simulink model "SC03_testbench"  (R2025a)
settings: Solver=ode23tb  StartTime=0.0  StopTime=52.6667  MaxStep=1e-5  RelTol=1e-4
InitFcn:
  | tbModel = 'SC03_testbench'; sc03_tb_init
model workspace (MAT data in the model file):
  tbGroup = 'bat'
values from neighbouring files (symbols this model uses):
  sw = swMap_(cfg)    [sc03_tb_init.m]
  useMem = double(cfg == 4)    [sc03_tb_init.m]
undefined symbols (not defined in the file or in its folder): Ion, Lithium, scen
libraries: spsSeriesRLCBranchLib x8, spsDiodeLib x4, spsPVArrayLib x4, simulink x3, spsCurrentMeasurementLib x2, fuzblock x2, spsBatteryLib x1, spsBuckConverterLib x1, spsGroundLib x1, spsVoltageMeasurementLib x1, sps_lib x1
settings Model: PauseTimes=8  Creator=kaush  LastModifiedBy=kaush
settings SolverCC: ZeroCrossAlgorithm=Adaptive  AlgebraicLoopSolver=TrustRegion
settings DataIOCC: SignalLogging=off
settings DebuggingCC: AlgebraicLoopMsg=none  IgnoredZcDiagnostic=none

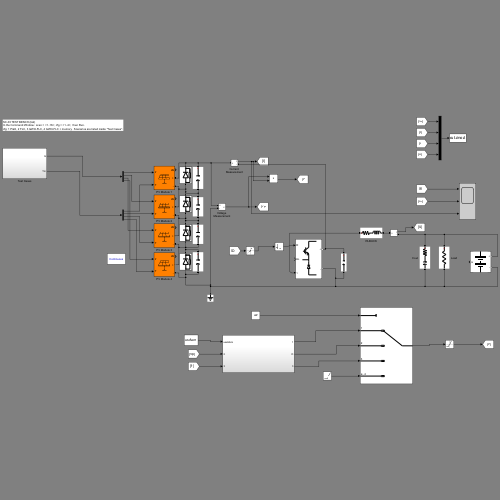
[thumbnail: Simulink's stored preview of the top-level diagram]
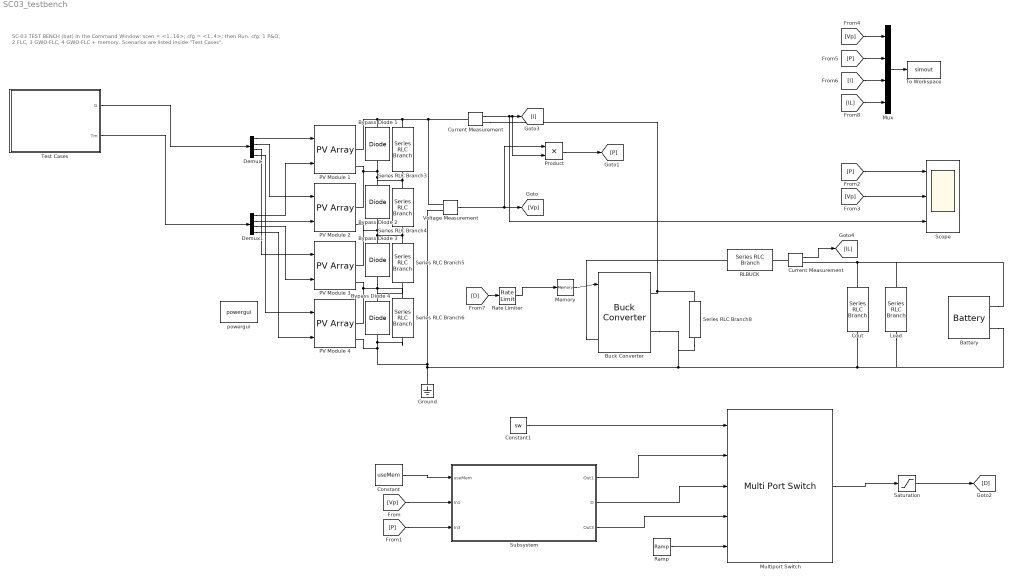
== system SC03_testbench ==
  note: SC-03 TEST BENCH (bat)
      | In the Command Window:  scen = <1..16>; cfg = <1..4>;  then Run.
      | cfg: 1 P&O, 2 FLC, 3 GWO-FLC, 4 GWO-FLC + memory.  Scenarios are listed inside "Test Cases".
  Battery : spsBatteryLib/Battery  BatType=Lithium-Ion  NomV=12.8  NomQ=160  SOC=55  Batt_Tr=30  PresetModel=off  MaxQ=160  MinV=11.2  FullV=14.4  Dis_rate=69.5652  R=0.0009  Normal_OP=144.6957  expZone="[13.8289      7.86087]"
  Buck Converter : spsBuckConverterLib/Buck Converter  ModelType=Average model (D-controlled)  Ron=1e-3  Rs=1e6  Cs=inf  Vforward=[0,0]  Ron_Diode=1e-3  Rs_Diode=1e6  Cs_Diode=inf  Vf_Diode=1e-3  Rs_CurrentSource=inf  Ron_ACsource=1e-3
      settings: LibrarySourceBlock=sps_lib/Power Electronics/Buck Converter
  Bypass Diode {1..4} (4 alike) : spsDiodeLib/Diode  Ron=0.001  Lon=0  Vf=0.8  IC=0  UseSnubber=off  Rs=500  Cs=250e-9  Measurements=off
  Constant : Constant  Value=useMem
  Constant1 : Constant  Value=sw
  Cout : spsSeriesRLCBranchLib/Series RLC Branch  LConnTagsString=__new0  RConnTagsString=__new0  BranchType=RC  Resistance=0.02  Inductance=1e-3  SetiL0=off  InitialCurrent=0  Capacitance=470e-6  Setx0=off  InitialVoltage=0  Measurements=None
  Current Measurement : spsCurrentMeasurementLib/Current Measurement  PhasorSimulation=off  OutputType=Complex  PSBequivalent=0
  Current Measurement : spsCurrentMeasurementLib/Current Measurement  PhasorSimulation=off  OutputType=Complex  PSBequivalent=0
  Demux : Demux
  Demux1 : Demux
  Ground : spsGroundLib/Ground  LConnTagsString=a
  Load : spsSeriesRLCBranchLib/Series RLC Branch  LConnTagsString=__new0  RConnTagsString=__new0  BranchType=R  Resistance=1.25  Inductance=1e-3  SetiL0=off  InitialCurrent=0  Capacitance=1000e-6  Setx0=on  InitialVoltage=33  Measurements=None
  Memory : Memory  InitialCondition=0.44
  Multiport Switch : MultiPortSwitch  Inputs=4  SaturateOnIntegerOverflow=off  InputSameDT=off
  Mux : Mux
  PV Module {1..4} (4 alike) : spsPVArrayLib/PV Array  Npar=1  Nser=1  PlotType=array @ 1000 W/m2 & specified temperatures  S_vec="[ 1000  500  100 ]"  Temp_C_vec="[ 45 25  ]"  ModuleName=User-defined  PlotWhenSelected=off  Pm=39.961  Ncell=18  Voc=11.15  Isc=4.85  Vm=8.9  Im=4.49  beta_Voc_pc=-0.35  alpha_Isc_pc=0.06  beta_Voc=-0.039025  alpha_Isc=0.00291  IL=4.8622  I0=1.1491e-10  nI=0.98652  Rsh=80.7946  Rs=0.20279  RobustModel=off  RobustCellTemperature=313.3991  BAL=off  Tc=1e-6  Tfilter=5e-5
  Product : Product
  RLBUCK : spsSeriesRLCBranchLib/Series RLC Branch  LConnTagsString=__new0  RConnTagsString=__new0  BranchType=RL  Resistance=0.03  Inductance=150e-6  SetiL0=off  InitialCurrent=0  Capacitance=220e-6  Setx0=off  InitialVoltage=0  Measurements=None
  Ramp : simulink/Sources/Ramp  slope=0.1  start=0.6  InitialOutput=0.2
  Rate Limiter : RateLimiter  RisingSlewLimit=50  FallingSlewLimit=-50
  Saturation : Saturate  UpperLimit=0.9  LowerLimit=0.2  OutDataTypeStr=double
  Scope : Scope  NumInputPorts=3
      settings: SampleTime=5e-3  ActiveDisplayYMinimum=-48.915122652738674  ActiveDisplayYMaximum=132.79135271459734  DataLoggingVariableName=ScopeData3
  Series RLC Branch{3..6} (4 alike) : spsSeriesRLCBranchLib/Series RLC Branch  LConnTagsString=__new0  RConnTagsString=__new0  BranchType=C  Resistance=1  Inductance=1e-3  SetiL0=off  InitialCurrent=0  Capacitance=1e-6  Setx0=off  InitialVoltage=0  Measurements=None
  Series RLC Branch8 : spsSeriesRLCBranchLib/Series RLC Branch  LConnTagsString=__new0  RConnTagsString=__new0  BranchType=C  Resistance=1  Inductance=1e-3  SetiL0=off  InitialCurrent=0  Capacitance=220e-6  Setx0=off  InitialVoltage=0  Measurements=None
  Subsystem : Subsystem
  Test Cases : Subsystem  Description=Set scen (1-16) and cfg (1-4) in the Command Window, then Run.
  To Workspace : ToWorkspace  VariableName=simout  SaveFormat=Timeseries  SampleTime=1e-3
  Voltage Measurement : spsVoltageMeasurementLib/Voltage Measurement  PhasorSimulation=off  OutputType=Complex  PSBequivalent=0
  powergui : sps_lib/powergui  Priority=1  SimulationMode=Continuous  SampleTime=50e-6  frequency=60  Iterations=50  frequencyindice=0  Pbase=100e6  ErrMax=1e-4  UnitsV=kV  UnitsW=MW  buscounter=0  FunctionMessages=off  echomessages=off  EnableUseOfTLC=off  CurrentSourceSwitches=off  DisableSnubberDevices=off  DisableRonSwitches=off  DisableVfSwitches=off  DisplayEquations=off  AutomaticDiscreteSolvers=off  SolverType=Tustin/Backward Euler (TBE)  Interpol=off  ExternalGateDelay=off  methode=off  Ts=100  x0status=blocks  SPID=off  SwTol=0  HookPort=off  NonlinearTolerance=1e-4  nMaxIteration=100  ContinueOnMaxIteration=off  RestoreLinks=warning  ResistiveCurrentMeasurement=off  Frange=[0:2:500]  Ylog=off  Xlog=on  ShowGrid=off  save=off  variable=ZData  structure=0  ZoomFFT=off  StartTime=0.0  cycles=1  DisplayStyle=1  fundamental=60  FreqAxis=off  MaxFrequency=1000  frequencyindicesteady=1  RmsSteady=1  display=off
  wires:
  Multiport Switch/1 -> Saturation/1
  [D] -> Rate Limiter/1
  Demux1/3 -> PV Module 3/2
  Memory/1 -> Buck Converter/1
  Mux/1 -> To Workspace/1
  Product/1 -> [P]
  Demux/2 -> PV Module 2/1
  Demux1/2 -> PV Module 2/2
  Current Measurement/1 -> Scope/3, Product/2, [I]
  Demux/4 -> PV Module 4/1
  Voltage Measurement/1 -> Product/1, [Vp]
  Demux/1 -> PV Module 1/1
  Demux/3 -> PV Module 3/1
  Demux1/1 -> PV Module 1/2
  Demux1/4 -> PV Module 4/2
  Constant/1 -> Subsystem/1(useMem)
  Subsystem/1(Out1) -> Multiport Switch/2
  Subsystem/2(D) -> Multiport Switch/3
  Subsystem/3(Out3) -> Multiport Switch/4
  Constant1/1 -> Multiport Switch/1
  [Vp] -> Subsystem/2(In1)
  [P] -> Subsystem/3(In3)
  [P] -> Scope/1
  [Vp] -> Scope/2
  [Vp] -> Mux/1
  [P] -> Mux/2
  [I] -> Mux/3
  Current Measurement/1 -> [IL]
  [IL] -> Mux/4
  Saturation/1 -> [D]
  Rate Limiter/1 -> Memory/1
  Ramp/1 -> Multiport Switch/5
  Test Cases/1(G) -> Demux/1
  Test Cases/2(Tm) -> Demux1/1
  connections:
  Cout/RConn1 -- Battery/LConn2 -- Load/RConn1 -- Buck Converter/RConn2 -- Series RLC Branch8/RConn1 -- Voltage Measurement/LConn2 -- PV Module 4/RConn2 -- Series RLC Branch6/RConn1 -- Bypass Diode 4/LConn1 -- Ground/LConn1
  Series RLC Branch8/LConn1 -- Current Measurement/RConn1 -- Buck Converter/RConn1
  PV Module 4/RConn1 -- PV Module 3/RConn2 -- Series RLC Branch6/LConn1 -- Bypass Diode 4/RConn1 -- Series RLC Branch5/RConn1 -- Bypass Diode 3/LConn1
  Series RLC Branch4/RConn1 -- Bypass Diode 2/LConn1 -- PV Module 3/RConn1 -- PV Module 2/RConn2 -- Bypass Diode 3/RConn1 -- Series RLC Branch5/LConn1
  Series RLC Branch3/RConn1 -- Bypass Diode 1/LConn1 -- PV Module 1/RConn2 -- PV Module 2/RConn1 -- Bypass Diode 2/RConn1 -- Series RLC Branch4/LConn1
  Current Measurement/LConn1 -- Voltage Measurement/LConn1 -- PV Module 1/RConn1 -- Bypass Diode 1/RConn1 -- Series RLC Branch3/LConn1
  Cout/LConn1 -- Battery/LConn1 -- Load/LConn1 -- Current Measurement/RConn1
  Current Measurement/LConn1 -- RLBUCK/RConn1
  RLBUCK/LConn1 -- Buck Converter/LConn1

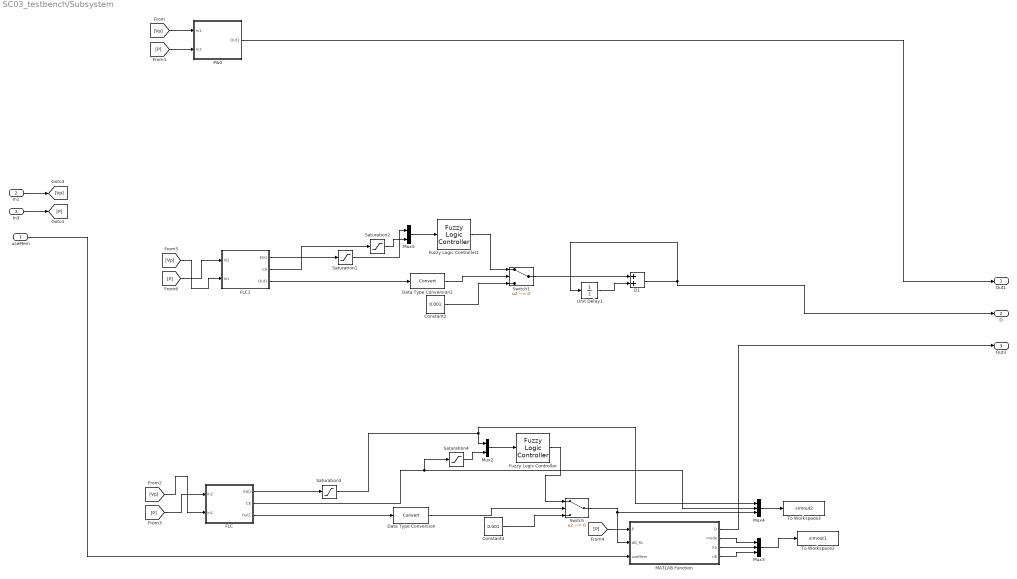
== system SC03_testbench/Subsystem ==
  useMem : Inport
  In1 : Inport  Port=2
  In3 : Inport  Port=3
  Constant2 : Constant  Value=0.001
  Constant4 : Constant  Value=0.001
  D1 : Sum
  Data Type Conversion : DataTypeConversion  SaturateOnIntegerOverflow=off  RndMeth=Floor
  Data Type Conversion1 : DataTypeConversion  SaturateOnIntegerOverflow=off  RndMeth=Floor
  FLC : Subsystem
  FLC1 : Subsystem
  Fuzzy Logic Controller : fuzblock/Fuzzy Logic  Controller  FIS='flc_mppt.fis'  OutputSampleNumber=101  DataType=double  UseLookupTable=off  NumBreakpoints=10  FuzzifiedInputs=off  RuleFiringStrengths=off  RuleOutputs=off  AggregatedOutputs=off  SimulateUsing=Interpreted execution  OutOfRangeInputValueMessage=warning  NoRuleFiredMessage=warning  EmptyOutputFuzzySetMessage=warning
  Fuzzy Logic Controller1 : fuzblock/Fuzzy Logic  Controller  FIS='flc_mppt.fis'  OutputSampleNumber=101  DataType=double  UseLookupTable=off  NumBreakpoints=10  FuzzifiedInputs=off  RuleFiringStrengths=off  RuleOutputs=off  AggregatedOutputs=off  SimulateUsing=Interpreted execution  OutOfRangeInputValueMessage=warning  NoRuleFiredMessage=warning  EmptyOutputFuzzySetMessage=warning
  MATLAB Function : MATLAB Function  TreatAsAtomicUnit=on
  Mux2 : Mux  Inputs=2
  Mux3 : Mux  Inputs=3
  Mux4 : Mux  Inputs=3
  Mux5 : Mux  Inputs=2
  P&0 : Subsystem  SystemSampleTime=5e-3
  Saturation1 : Saturate  UpperLimit=4.75  LowerLimit=-32
  Saturation2 : Saturate  UpperLimit=6  LowerLimit=-6
  Saturation3 : Saturate  UpperLimit=4.75  LowerLimit=-32
  Saturation4 : Saturate  UpperLimit=6  LowerLimit=-6
  Switch : Switch  Criteria=u2 ~= 0  SaturateOnIntegerOverflow=off  InputSameDT=off
  Switch1 : Switch  Criteria=u2 ~= 0  SaturateOnIntegerOverflow=off  InputSameDT=off
  To Workspace2 : ToWorkspace  VariableName=simout1  SaveFormat=Timeseries  SampleTime=-1
  To Workspace3 : ToWorkspace  VariableName=simout2  SaveFormat=Timeseries  SampleTime=0.03
  Unit Delay1 : UnitDelay  InitialCondition=0.44  SampleTime=0.03  HasFrameUpgradeWarning=on
  Out1 : Outport
  D : Outport  Port=2
  Out3 : Outport  Port=3
  wires:
  D1/1 -> D/1, Unit Delay1/1
  Unit Delay1/1 -> D1/2
  P&0/1(Out1) -> Out1/1
  FLC1/2(CE) -> Saturation2/1
  Switch/1 -> Mux4/3, MATLAB Function/2(dD_flc)
  FLC1/3(Out1) -> Data Type Conversion1/1
  Switch1/1 -> D1/1
  [P] -> FLC1/1(In2)
  Fuzzy Logic Controller1/1 -> Switch1/1
  Constant2/1 -> Switch1/3
  [P] -> MATLAB Function/1(P)
  [Vp] -> FLC1/2(In1)
  Saturation2/1 -> Mux5/2
  Fuzzy Logic Controller/1 -> Switch/1
  Saturation4/1 -> Mux2/2
  FLC1/1(E(K)) -> Saturation1/1
  Data Type Conversion1/1 -> Switch1/2
  Saturation1/1 -> Mux5/1
  Mux5/1 -> Fuzzy Logic Controller1/1
  Saturation3/1 -> Mux4/1, Mux2/1
  FLC/1(E(K)) -> Saturation3/1
  Data Type Conversion/1 -> Switch/2
  MATLAB Function/2(mode) -> Mux3/1
  MATLAB Function/4(nE) -> Mux3/3
  MATLAB Function/3(Xa) -> Mux3/2
  Constant4/1 -> Switch/3
  Mux3/1 -> To Workspace2/1
  Mux2/1 -> Fuzzy Logic Controller/1
  Mux4/1 -> To Workspace3/1
  FLC/2(CE) -> Saturation4/1, Mux4/2
  FLC/3(Out1) -> Data Type Conversion/1
  MATLAB Function/1(D) -> Out3/1
  useMem/1 -> MATLAB Function/3(useMem)
  In1/1 -> [Vp]
  In3/1 -> [P]
  [Vp] -> P&0/1(In1)
  [P] -> P&0/2(In2)
  [Vp] -> FLC/2(In1)
  [P] -> FLC/1(In2)

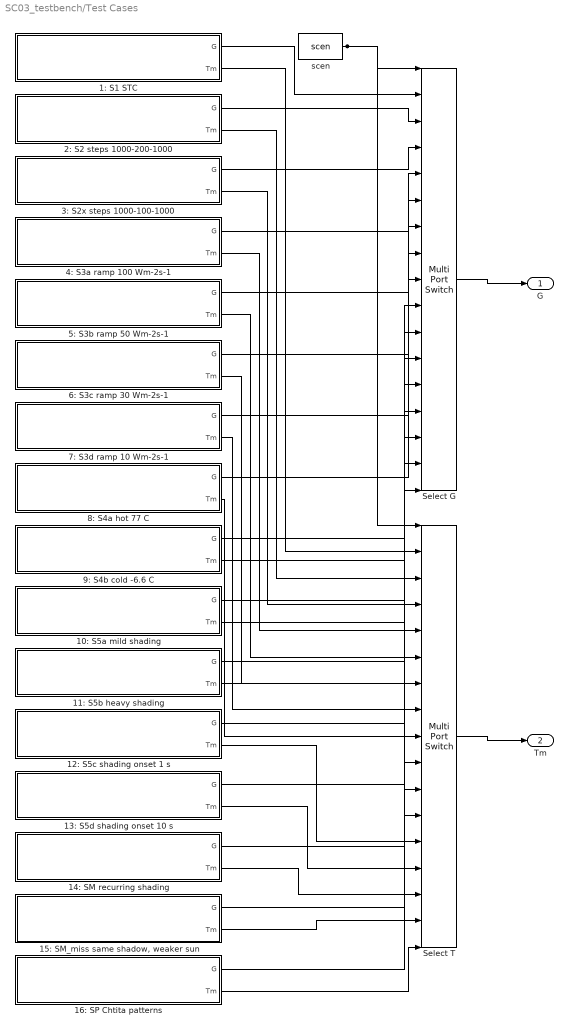
== system SC03_testbench/Test Cases ==
  10: S5a mild shading : Subsystem  Description=Stop time 4 s, module temperature 25 C
  11: S5b heavy shading : Subsystem  Description=Stop time 4 s, module temperature 25 C
  12: S5c shading onset 1 s : Subsystem  Description=Stop time 6 s, module temperature 25 C
  13: S5d shading onset 10 s : Subsystem  Description=Stop time 16 s, module temperature 25 C
  14: SM recurring shading : Subsystem  Description=Stop time 8 s, module temperature 25 C
  "15: SM_miss same shadow, weaker sun" : Subsystem  Description=Stop time 8 s, module temperature 25 C
  16: SP Chtita patterns : Subsystem  Description=Stop time 8 s, module temperature 25 C
  1: S1 STC : Subsystem  Description=Stop time 3 s, module temperature 25 C
  2: S2 steps 1000-200-1000 : Subsystem  Description=Stop time 6 s, module temperature 25 C
  3: S2x steps 1000-100-1000 : Subsystem  Description=Stop time 6 s, module temperature 25 C
  4: S3a ramp 100 Wm-2s-1 : Subsystem  Description=Stop time 20 s, module temperature 25 C
  5: S3b ramp 50 Wm-2s-1 : Subsystem  Description=Stop time 22 s, module temperature 25 C
  6: S3c ramp 30 Wm-2s-1 : Subsystem  Description=Stop time 52.6667 s, module temperature 25 C
  7: S3d ramp 10 Wm-2s-1 : Subsystem  Description=Stop time 146 s, module temperature 25 C
  8: S4a hot 77 C : Subsystem  Description=Stop time 3 s, module temperature 77 C
  9: S4b cold -6.6 C : Subsystem  Description=Stop time 3 s, module temperature -6.6 C
  Select G : MultiPortSwitch  Inputs=16  SaturateOnIntegerOverflow=off  InputSameDT=off
  Select T : MultiPortSwitch  Inputs=16  SaturateOnIntegerOverflow=off  InputSameDT=off
  scen : Constant  Value=scen
  G : Outport
  Tm : Outport  Port=2
  wires:
  scen/1 -> Select G/1, Select T/1
  Select G/1 -> G/1
  Select T/1 -> Tm/1
  1: S1 STC/1(G) -> Select G/2
  1: S1 STC/2(Tm) -> Select T/2
  2: S2 steps 1000-200-1000/1(G) -> Select G/3
  2: S2 steps 1000-200-1000/2(Tm) -> Select T/3
  3: S2x steps 1000-100-1000/1(G) -> Select G/4
  3: S2x steps 1000-100-1000/2(Tm) -> Select T/4
  4: S3a ramp 100 Wm-2s-1/1(G) -> Select G/5
  4: S3a ramp 100 Wm-2s-1/2(Tm) -> Select T/5
  5: S3b ramp 50 Wm-2s-1/1(G) -> Select G/6
  5: S3b ramp 50 Wm-2s-1/2(Tm) -> Select T/6
  6: S3c ramp 30 Wm-2s-1/1(G) -> Select G/7
  6: S3c ramp 30 Wm-2s-1/2(Tm) -> Select T/7
  7: S3d ramp 10 Wm-2s-1/1(G) -> Select G/8
  7: S3d ramp 10 Wm-2s-1/2(Tm) -> Select T/8
  8: S4a hot 77 C/1(G) -> Select G/9
  8: S4a hot 77 C/2(Tm) -> Select T/9
  9: S4b cold -6.6 C/1(G) -> Select G/10
  9: S4b cold -6.6 C/2(Tm) -> Select T/10
  10: S5a mild shading/1(G) -> Select G/11
  10: S5a mild shading/2(Tm) -> Select T/11
  11: S5b heavy shading/1(G) -> Select G/12
  11: S5b heavy shading/2(Tm) -> Select T/12
  12: S5c shading onset 1 s/1(G) -> Select G/13
  12: S5c shading onset 1 s/2(Tm) -> Select T/13
  13: S5d shading onset 10 s/1(G) -> Select G/14
  13: S5d shading onset 10 s/2(Tm) -> Select T/14
  14: SM recurring shading/1(G) -> Select G/15
  14: SM recurring shading/2(Tm) -> Select T/15
  "15: SM_miss same shadow, weaker sun"/1(G) -> Select G/16
  "15: SM_miss same shadow, weaker sun"/2(Tm) -> Select T/16
  16: SP Chtita patterns/1(G) -> Select G/17
  16: SP Chtita patterns/2(Tm) -> Select T/17

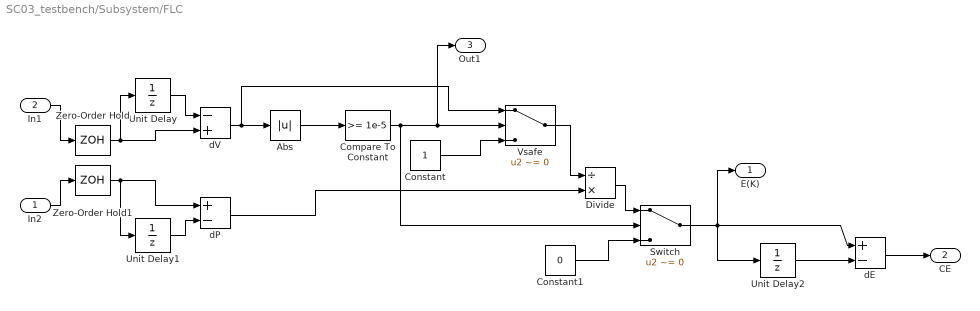
== system SC03_testbench/Subsystem/FLC ==
  In2 : Inport
  In1 : Inport  Port=2
  Abs : Abs  SaturateOnIntegerOverflow=off
  Compare To Constant : simulink/Logic and Bit Operations/Compare To Constant  relop=>=  const=1e-5  OutDataTypeStr=boolean
  Constant : Constant
  Constant1 : Constant  Value=0
  Divide : Product  Inputs=/*
  Switch : Switch  Criteria=u2 ~= 0  SaturateOnIntegerOverflow=off  InputSameDT=off
  Unit Delay : UnitDelay  SampleTime=-1  HasFrameUpgradeWarning=on
  Unit Delay1 : UnitDelay  SampleTime=-1  HasFrameUpgradeWarning=on
  Unit Delay2 : UnitDelay  SampleTime=-1  HasFrameUpgradeWarning=on
  Vsafe : Switch  Criteria=u2 ~= 0  SaturateOnIntegerOverflow=off  InputSameDT=off
  Zero-Order Hold : ZeroOrderHold  SampleTime=0.03
  Zero-Order Hold1 : ZeroOrderHold  SampleTime=0.03
  dE : Sum  Inputs=+-
  dP : Sum  Inputs=+-
  dV : Sum  Inputs=-+
  E(K) : Outport
  CE : Outport  Port=2
  Out1 : Outport  Port=3
  wires:
  dV/1 -> Vsafe/1, Abs/1
  Unit Delay1/1 -> dP/2
  In1/1 -> Zero-Order Hold/1
  In2/1 -> Zero-Order Hold1/1
  Unit Delay/1 -> dV/1
  Zero-Order Hold1/1 -> Unit Delay1/1, dP/1
  Zero-Order Hold/1 -> dV/2, Unit Delay/1
  Abs/1 -> Compare To Constant/1
  Compare To Constant/1 -> Switch/2, Out1/1, Vsafe/2
  Constant/1 -> Vsafe/3
  dP/1 -> Divide/2
  Vsafe/1 -> Divide/1
  Divide/1 -> Switch/1
  Constant1/1 -> Switch/3
  Unit Delay2/1 -> dE/2
  Switch/1 -> dE/1, Unit Delay2/1, E(K)/1
  dE/1 -> CE/1

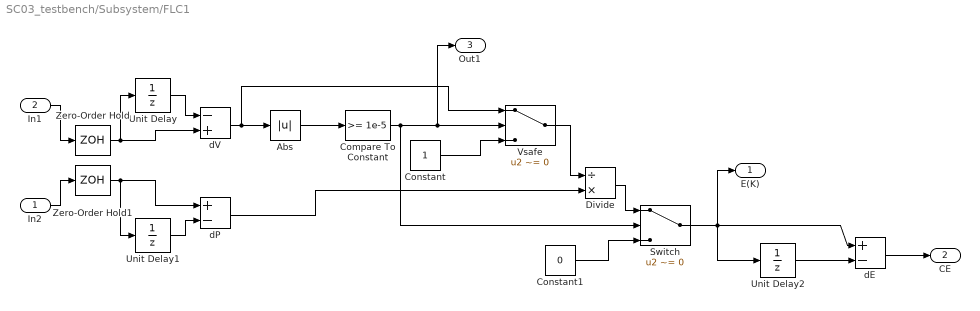
== system SC03_testbench/Subsystem/FLC1 ==
  In2 : Inport
  In1 : Inport  Port=2
  Abs : Abs  SaturateOnIntegerOverflow=off
  Compare To Constant : simulink/Logic and Bit Operations/Compare To Constant  relop=>=  const=1e-5  OutDataTypeStr=boolean
  Constant : Constant
  Constant1 : Constant  Value=0
  Divide : Product  Inputs=/*
  Switch : Switch  Criteria=u2 ~= 0  SaturateOnIntegerOverflow=off  InputSameDT=off
  Unit Delay : UnitDelay  SampleTime=-1  HasFrameUpgradeWarning=on
  Unit Delay1 : UnitDelay  SampleTime=-1  HasFrameUpgradeWarning=on
  Unit Delay2 : UnitDelay  SampleTime=-1  HasFrameUpgradeWarning=on
  Vsafe : Switch  Criteria=u2 ~= 0  SaturateOnIntegerOverflow=off  InputSameDT=off
  Zero-Order Hold : ZeroOrderHold  SampleTime=0.03
  Zero-Order Hold1 : ZeroOrderHold  SampleTime=0.03
  dE : Sum  Inputs=+-
  dP : Sum  Inputs=+-
  dV : Sum  Inputs=-+
  E(K) : Outport
  CE : Outport  Port=2
  Out1 : Outport  Port=3
  wires:
  dV/1 -> Vsafe/1, Abs/1
  Unit Delay1/1 -> dP/2
  In1/1 -> Zero-Order Hold/1
  In2/1 -> Zero-Order Hold1/1
  Unit Delay/1 -> dV/1
  Zero-Order Hold1/1 -> Unit Delay1/1, dP/1
  Zero-Order Hold/1 -> dV/2, Unit Delay/1
  Abs/1 -> Compare To Constant/1
  Compare To Constant/1 -> Switch/2, Out1/1, Vsafe/2
  Constant/1 -> Vsafe/3
  dP/1 -> Divide/2
  Vsafe/1 -> Divide/1
  Divide/1 -> Switch/1
  Constant1/1 -> Switch/3
  Unit Delay2/1 -> dE/2
  Switch/1 -> dE/1, Unit Delay2/1, E(K)/1
  dE/1 -> CE/1

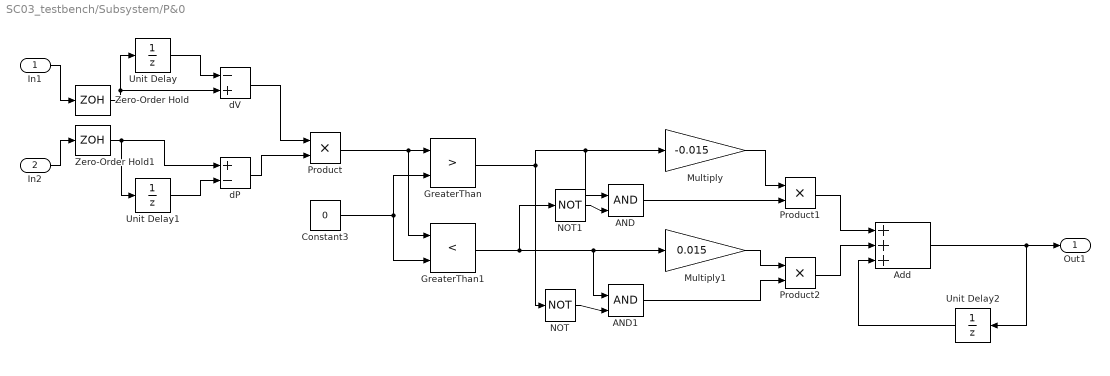
== system SC03_testbench/Subsystem/P&0 ==
  In1 : Inport
  In2 : Inport  Port=2
  AND : Logic  IconShape=distinctive  AllPortsSameDT=off  OutDataTypeStr=boolean
  AND1 : Logic  IconShape=distinctive  AllPortsSameDT=off  OutDataTypeStr=boolean
  Add : Sum  Inputs=+++
  Constant3 : Constant  Value=0
  GreaterThan : RelationalOperator  Operator=>  OutDataTypeStr=boolean  RndMeth=Simplest  InputSameDT=off
  GreaterThan1 : RelationalOperator  Operator=<  OutDataTypeStr=boolean  RndMeth=Simplest  InputSameDT=off
  Multiply : Gain  Gain=-0.015
  Multiply1 : Gain  Gain=0.015
  NOT : Logic  Operator=NOT  IconShape=distinctive  AllPortsSameDT=off  OutDataTypeStr=boolean
  NOT1 : Logic  Operator=NOT  IconShape=distinctive  AllPortsSameDT=off  OutDataTypeStr=boolean
  Product : Product
  Product1 : Product  OutDataTypeStr=double
  Product2 : Product  OutDataTypeStr=double
  Unit Delay : UnitDelay  SampleTime=-1  HasFrameUpgradeWarning=on
  Unit Delay1 : UnitDelay  SampleTime=-1  HasFrameUpgradeWarning=on
  Unit Delay2 : UnitDelay  InitialCondition=0.44  SampleTime=0.03  HasFrameUpgradeWarning=on
  Zero-Order Hold : ZeroOrderHold  SampleTime=0.03
  Zero-Order Hold1 : ZeroOrderHold  SampleTime=0.03
  dP : Sum  Inputs=+-
  dV : Sum  Inputs=-+
  Out1 : Outport
  wires:
  dV/1 -> Product/1
  Multiply1/1 -> Product2/1
  Unit Delay1/1 -> dP/2
  Add/1 -> Out1/1, Unit Delay2/1
  GreaterThan1/1 -> NOT1/1, Multiply1/1, AND1/1
  In1/1 -> Zero-Order Hold/1
  In2/1 -> Zero-Order Hold1/1
  Unit Delay/1 -> dV/1
  Constant3/1 -> GreaterThan/2, GreaterThan1/2
  AND/1 -> Product1/2
  AND1/1 -> Product2/2
  GreaterThan/1 -> Multiply/1, AND/1, NOT/1
  Multiply/1 -> Product1/1
  NOT1/1 -> AND/2
  Product/1 -> GreaterThan1/1, GreaterThan/1
  dP/1 -> Product/2
  Product1/1 -> Add/1
  Unit Delay2/1 -> Add/3
  NOT/1 -> AND1/2
  Product2/1 -> Add/2
  Zero-Order Hold1/1 -> Unit Delay1/1, dP/1
  Zero-Order Hold/1 -> dV/2, Unit Delay/1

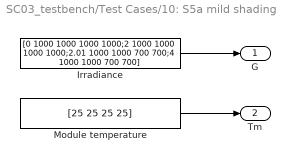
== system SC03_testbench/Test Cases/10: S5a mild shading ==
  Irradiance : FromWorkspace  VariableName=[0 1000 1000 1000 1000;2 1000 1000 1000 1000;2.01 1000 1000 700 700;4 1000 1000 700 700]  OutputAfterFinalValue=Holding final value
  Module temperature : Constant  Value=[25 25 25 25]
  G : Outport
  Tm : Outport  Port=2
  wires:
  Irradiance/1 -> G/1
  Module temperature/1 -> Tm/1

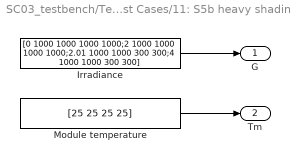
== system SC03_testbench/Test Cases/11: S5b heavy shading ==
  Irradiance : FromWorkspace  VariableName=[0 1000 1000 1000 1000;2 1000 1000 1000 1000;2.01 1000 1000 300 300;4 1000 1000 300 300]  OutputAfterFinalValue=Holding final value
  Module temperature : Constant  Value=[25 25 25 25]
  G : Outport
  Tm : Outport  Port=2
  wires:
  Irradiance/1 -> G/1
  Module temperature/1 -> Tm/1

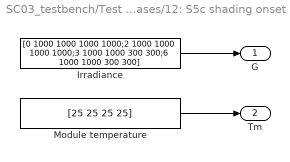
== system SC03_testbench/Test Cases/12: S5c shading onset 1 s ==
  Irradiance : FromWorkspace  VariableName=[0 1000 1000 1000 1000;2 1000 1000 1000 1000;3 1000 1000 300 300;6 1000 1000 300 300]  OutputAfterFinalValue=Holding final value
  Module temperature : Constant  Value=[25 25 25 25]
  G : Outport
  Tm : Outport  Port=2
  wires:
  Irradiance/1 -> G/1
  Module temperature/1 -> Tm/1

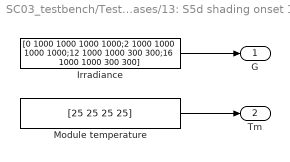
== system SC03_testbench/Test Cases/13: S5d shading onset 10 s ==
  Irradiance : FromWorkspace  VariableName=[0 1000 1000 1000 1000;2 1000 1000 1000 1000;12 1000 1000 300 300;16 1000 1000 300 300]  OutputAfterFinalValue=Holding final value
  Module temperature : Constant  Value=[25 25 25 25]
  G : Outport
  Tm : Outport  Port=2
  wires:
  Irradiance/1 -> G/1
  Module temperature/1 -> Tm/1

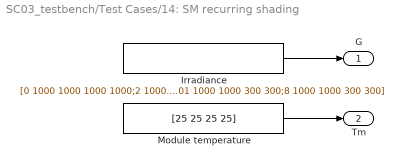
== system SC03_testbench/Test Cases/14: SM recurring shading ==
  Irradiance : FromWorkspace  VariableName=[0 1000 1000 1000 1000;2 1000 1000 1000 1000;2.01 1000 1000 300 300;4 1000 1000 300 300;4.01 1000 1000 1000 1000;6 1000 1000 1000 1000;6.01 1000 1000 300 300;8 1000 1000 300 300]  OutputAfterFinalValue=Holding final value
  Module temperature : Constant  Value=[25 25 25 25]
  G : Outport
  Tm : Outport  Port=2
  wires:
  Irradiance/1 -> G/1
  Module temperature/1 -> Tm/1

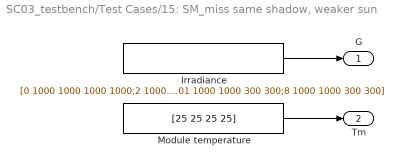
== system SC03_testbench/Test Cases/15: SM_miss same shadow, weaker sun ==
  Irradiance : FromWorkspace  VariableName=[0 1000 1000 1000 1000;2 1000 1000 1000 1000;2.01 1000 1000 300 300;4 1000 1000 300 300;4.01 700 700 210 210;6 700 700 210 210;6.01 1000 1000 300 300;8 1000 1000 300 300]  OutputAfterFinalValue=Holding final value
  Module temperature : Constant  Value=[25 25 25 25]
  G : Outport
  Tm : Outport  Port=2
  wires:
  Irradiance/1 -> G/1
  Module temperature/1 -> Tm/1

== system SC03_testbench/Test Cases/16: SP Chtita patterns ==
  Irradiance : FromWorkspace  VariableName=[0 1000 1000 1000 1000;2 1000 1000 1000 1000;2.01 1000 700 100 1000;4 1000 700 100 1000;4.01 1000 500 1000 1000;6 1000 500 1000 1000;6.01 1000 700 500 250;8 1000 700 500 250]  OutputAfterFinalValue=Holding final value
  Module temperature : Constant  Value=[25 25 25 25]
  G : Outport
  Tm : Outport  Port=2
  wires:
  Irradiance/1 -> G/1
  Module temperature/1 -> Tm/1

== system SC03_testbench/Test Cases/1: S1 STC ==
  Irradiance : FromWorkspace  VariableName=[0 1000 1000 1000 1000;3 1000 1000 1000 1000]  OutputAfterFinalValue=Holding final value
  Module temperature : Constant  Value=[25 25 25 25]
  G : Outport
  Tm : Outport  Port=2
  wires:
  Irradiance/1 -> G/1
  Module temperature/1 -> Tm/1

== system SC03_testbench/Test Cases/2: S2 steps 1000-200-1000 ==
  Irradiance : FromWorkspace  VariableName=[0 1000 1000 1000 1000;2 1000 1000 1000 1000;2.01 200 200 200 200;4 200 200 200 200;4.01 1000 1000 1000 1000;6 1000 1000 1000 1000]  OutputAfterFinalValue=Holding final value
  Module temperature : Constant  Value=[25 25 25 25]
  G : Outport
  Tm : Outport  Port=2
  wires:
  Irradiance/1 -> G/1
  Module temperature/1 -> Tm/1

== system SC03_testbench/Test Cases/3: S2x steps 1000-100-1000 ==
  Irradiance : FromWorkspace  VariableName=[0 1000 1000 1000 1000;2 1000 1000 1000 1000;2.01 100 100 100 100;4 100 100 100 100;4.01 1000 1000 1000 1000;6 1000 1000 1000 1000]  OutputAfterFinalValue=Holding final value
  Module temperature : Constant  Value=[25 25 25 25]
  G : Outport
  Tm : Outport  Port=2
  wires:
  Irradiance/1 -> G/1
  Module temperature/1 -> Tm/1

== system SC03_testbench/Test Cases/4: S3a ramp 100 Wm-2s-1 ==
  Irradiance : FromWorkspace  VariableName=[0 1000 1000 1000 1000;2 1000 1000 1000 1000;9 300 300 300 300;11 300 300 300 300;18 1000 1000 1000 1000;20 1000 1000 1000 1000]  OutputAfterFinalValue=Holding final value
  Module temperature : Constant  Value=[25 25 25 25]
  G : Outport
  Tm : Outport  Port=2
  wires:
  Irradiance/1 -> G/1
  Module temperature/1 -> Tm/1

== system SC03_testbench/Test Cases/5: S3b ramp 50 Wm-2s-1 ==
  Irradiance : FromWorkspace  VariableName=[0 500 500 500 500;2 500 500 500 500;10 100 100 100 100;12 100 100 100 100;20 500 500 500 500;22 500 500 500 500]  OutputAfterFinalValue=Holding final value
  Module temperature : Constant  Value=[25 25 25 25]
  G : Outport
  Tm : Outport  Port=2
  wires:
  Irradiance/1 -> G/1
  Module temperature/1 -> Tm/1

== system SC03_testbench/Test Cases/6: S3c ramp 30 Wm-2s-1 ==
  Irradiance : FromWorkspace  VariableName=[0 1000 1000 1000 1000;2 1000 1000 1000 1000;25.333333 300 300 300 300;27.333333 300 300 300 300;50.666667 1000 1000 1000 1000;52.666667 1000 1000 1000 1000]  OutputAfterFinalValue=Holding final value
  Module temperature : Constant  Value=[25 25 25 25]
  G : Outport
  Tm : Outport  Port=2
  wires:
  Irradiance/1 -> G/1
  Module temperature/1 -> Tm/1

== system SC03_testbench/Test Cases/7: S3d ramp 10 Wm-2s-1 ==
  Irradiance : FromWorkspace  VariableName=[0 1000 1000 1000 1000;2 1000 1000 1000 1000;72 300 300 300 300;74 300 300 300 300;144 1000 1000 1000 1000;146 1000 1000 1000 1000]  OutputAfterFinalValue=Holding final value
  Module temperature : Constant  Value=[25 25 25 25]
  G : Outport
  Tm : Outport  Port=2
  wires:
  Irradiance/1 -> G/1
  Module temperature/1 -> Tm/1

== system SC03_testbench/Test Cases/8: S4a hot 77 C ==
  Irradiance : FromWorkspace  VariableName=[0 1000 1000 1000 1000;3 1000 1000 1000 1000]  OutputAfterFinalValue=Holding final value
  Module temperature : Constant  Value=[77 77 77 77]
  G : Outport
  Tm : Outport  Port=2
  wires:
  Irradiance/1 -> G/1
  Module temperature/1 -> Tm/1

== system SC03_testbench/Test Cases/9: S4b cold -6.6 C ==
  Irradiance : FromWorkspace  VariableName=[0 1000 1000 1000 1000;3 1000 1000 1000 1000]  OutputAfterFinalValue=Holding final value
  Module temperature : Constant  Value=[-6.6 -6.6 -6.6 -6.6]
  G : Outport
  Tm : Outport  Port=2
  wires:
  Irradiance/1 -> G/1
  Module temperature/1 -> Tm/1

== matlab function SC03_testbench/Subsystem/MATLAB Function ==
  settings: updateMethod=DISCRETE  sampleTime=0.03
  data: P input; D output; dD_flc input; mode output; Xa output; nE output; useMem input
function [D, mode, Xa, nE] = gwo_mppt(P, dD_flc, useMem)
%GWO_MPPT  Hybrid Grey Wolf Optimiser + Fuzzy Logic MPPT with a stored-peak memory.
%
%  WHAT IT DOES
%  The block runs once every Ta = 30 ms (set the block's sample time to 0.03).
%  Each call it receives the PV power P measured with the duty cycle it applied
%  on the previous call, and returns the next duty cycle D for the buck converter.
%
%  It works as a state machine with five states:
%    0  WAIT    - hold D for 0.6 s while the battery model settles
%    1  INIT    - place the wolves across the whole duty range
%    2  GWO     - global search: try one wolf per sample, move the pack each iteration
%    3  FLC     - local fine-tracking: add the fuzzy controller's step dD_flc to D
%    4  MEMORY  - after a shading change, try previously found peaks before searching
%
%  INPUTS   P       PV power [W] (sampled at this call)
%           dD_flc  duty step proposed by the fuzzy controller (used only in state 3)
%           useMem  0 = config C (plain GWO-FLC), 1 = config D (with memory)
%  OUTPUTS  D       duty cycle sent to the converter (via the Memory block)
%           mode    current state (logged to see what the controller is doing)
%           Xa      position of the alpha wolf (logged)
%           nE      running count of evaluations, i.e. samples spent testing points (logged)
%
%  SOURCES
%  GWO update: Mirjalili et al. (2014) and the author's reference code GWO.m v1.0.
%  One wolf per sample on a single converter: Mohanty et al. (2016).
%  GWO->FLC handover (Eq. 12, 2 %) and FLC->GWO restart (Eq. 13, 5 %): Eltamaly & Farh (2019).
%  Restart modified (own design): an absolute floor DPMIN is added to Eq. 13 and the first
%  FLC sample after a handover is not compared (see state 3).
%  Memory check and stored-wolf seeding: own design.

% ----------------------------------------------------------------------------------
% Tuning constants
% ----------------------------------------------------------------------------------
Dmin  = 0.20;  Dmax = 0.9;   % duty limits, identical for every controller
NW    = 4;                    % wolves in the pack
MAXIT = 8;                   % hard limit on GWO iterations per search
NWAIT = 20;                   % 20 samples x 30 ms = 0.6 s battery initialisation
EPS1  = 0.02;                 % Eq. 12: stop searching once alpha improves by < 2 %
EPS2  = 0.05;                 % Eq. 13: a >= 5 % power jump means the shading has changed
DPMIN = 3.2;                  % ...and the jump must also be >= 3.2 W (2 % of P_STC = 159.84 W)
MEMN  = 3;                    % memory remembers the last 3 global peaks
TOLM  = 0.02;                 % a stored peak "matches" if its power is within 2 %

% ----------------------------------------------------------------------------------
% Controller memory between calls. 'persistent' variables keep their value from
% one 30 ms call to the next, which is how the state machine remembers where it is.
% They are initialised once, on the very first call.
% ----------------------------------------------------------------------------------
persistent st cnt Dc Pos idx it Fa Fb Fd Xal Xbe Xde PaPrev Pprev seed nEval MemD MemP memN mi
if isempty(st)
    st = 0; cnt = 0; Dc = 0.44;               % start in WAIT, holding D = 0.44
    Pos = zeros(1,NW); idx = 1; it = 0;       % wolf positions, current wolf, iteration count
    Fa = inf; Fb = inf; Fd = inf;             % leader fitness values (see note in state 2)
    Xal = 0.44; Xbe = 0.44; Xde = 0.44;       % leader positions alpha, beta, delta
    PaPrev = 0; Pprev = 0;                    % previous powers for Eq. 12 and Eq. 13
    seed = 12345;                             % fixed seed -> identical random numbers every run
    nEval = 0;                                % evaluation counter (performance metric)
    MemD = zeros(1,MEMN); MemP = zeros(1,MEMN); memN = 0; mi = 1;   % empty memory
end

switch st

  % ================================================================================
  % STATE 0 - WAIT
  % The battery block's voltage drifts for the first ~0.5 s of every simulation.
  % Searching during that drift would give misleading power readings, so the
  % controller simply holds D = 0.44 for 0.6 s.
  % ================================================================================
  case 0
    cnt = cnt + 1;
    if cnt >= NWAIT, st = 1; end

  % ================================================================================
  % STATE 1 - INITIALISE THE PACK
  % Four wolves are placed at the centres of the four quarters of [0.31, 0.90], so the
  % first iteration samples the whole P-D curve and no peak can hide between them.
  % Fixed (rather than random) starting points make every run repeatable.
  %
  % Config D only: if a peak has been stored before, the fixed wolf closest to the
  % most recent stored peak is replaced by that stored duty ("seeding"). If the new
  % shading is similar to an old one, the pack starts with a wolf already near the
  % right peak; the other three still cover the rest of the range.
  % ================================================================================
  case 1
        Pos = [0.38 0.53 0.68 0.83];                 % quarter-centres of the feasible range [0.31, 0.90]
    idx = 1; it = 0; PaPrev = 0;
    if useMem > 0.5 && memN > 0
        [~, jn] = min(abs(Pos - MemD(1)));
        Pos(jn) = MemD(1);
    end
    Pos = sort(Pos, 'ascend');                  % evaluate low -> high (smallest duty jumps)
    Fa = inf; Fb = inf; Fd = inf;             % new shading = new curve, so forget old leaders
    Xal = Pos(1); Xbe = Pos(1); Xde = Pos(1);
    Dc = Pos(1);                              % apply wolf 1; it is measured on the next call
    st = 2;

  % ================================================================================
  % STATE 2 - GWO GLOBAL SEARCH
  % The converter can only sit at one duty at a time, so wolves are tested one per
  % sample: apply a wolf's duty, wait one Ta, read P on the next call.
  %
  % Leaders: alpha, beta and delta are the three best duties found so far in this
  % search. The reference code minimises, so fitness is f = -P (highest power =
  % lowest f). The three 'if' lines are copied from GWO.m lines 45-58.
  %
  % After all four wolves have been tested (one iteration):
  %   - Eltamaly & Farh Eq. 12: if alpha's power improved by less than 2 % since the
  %     last iteration (and at least 2 iterations have run), the right peak has been
  %     found -> jump to alpha and hand over to the FLC. The result is stored in memory.
  %   - otherwise every wolf moves towards a point guided by alpha, beta and delta
  %     (Mirjalili eqs. 3.3-3.7). The coefficient 'a' shrinks from 2 to 0 over the
  %     iterations: early on wolves can jump past the leaders (exploration), later
  %     they settle between them (convergence). New positions are clamped to the
  %     duty limits.
  % ================================================================================
  case 2
    nEval = nEval + 1;
    f = -P;
    if f < Fa,                     Fa = f; Xal = Pos(idx); end   % best so far   -> alpha
    if f > Fa && f < Fb,           Fb = f; Xbe = Pos(idx); end   % second best   -> beta
    if f > Fa && f > Fb && f < Fd, Fd = f; Xde = Pos(idx); end   % third best    -> delta
    idx = idx + 1;

    if idx <= NW                              % more wolves to test in this iteration
        Dc = Pos(idx);
    else                                      % iteration finished
        it = it + 1;
        Pa = -Fa;                             % alpha's power in watts

        if (it >= 2 && abs(Pa - PaPrev) <= EPS1*Pa) || it >= MAXIT
            % --- converged: hand over to the FLC at alpha ---
            % Pprev = 0: alpha's power Pa was measured up to two iterations ago, and during
            % an irradiance ramp it is out of date. The first FLC sample is therefore not
            % compared; it becomes the new reference for the restart check.
            Dc = Xal; Pprev = 0; st = 3;

            % --- store (D, P) of this peak. An entry counts as the same peak only if BOTH its
            %     duty (within 0.02) and its power (within TOLM) match; then its power is refreshed.
            %     Otherwise the peak is stored as a new entry, so a dimmer version of a stored
            %     shading pattern (same duty, lower power) cannot overwrite the original. ---
            j = 0;
            for k = 1:memN
                if abs(MemD(k) - Xal) < 0.02 && abs(MemP(k) - Pa) <= TOLM*Pa, j = k; end
            end
            if j > 0
                MemP(j) = Pa;
            else                              % newest peak goes first, oldest drops off
                MemD = [Xal MemD(1:MEMN-1)];
                MemP = [Pa  MemP(1:MEMN-1)];
                memN = min(memN + 1, MEMN);
            end

        else
            % --- not converged: move the pack (Mirjalili eqs. 3.3-3.7) ---
            PaPrev = Pa;
            a = 2 - (it-1)*(2/MAXIT);         % linearly decreasing from 2 towards 0
            for i = 1:NW
                % pull towards alpha
                [r1,seed] = lcg(seed); [r2,seed] = lcg(seed);
                A1 = 2*a*r1 - a;  C1 = 2*r2;
                X1 = Xal - A1*abs(C1*Xal - Pos(i));
                % pull towards beta
                [r1,seed] = lcg(seed); [r2,seed] = lcg(seed);
                A2 = 2*a*r1 - a;  C2 = 2*r2;
                X2 = Xbe - A2*abs(C2*Xbe - Pos(i));
                % pull towards delta
                [r1,seed] = lcg(seed); [r2,seed] = lcg(seed);
                A3 = 2*a*r1 - a;  C3 = 2*r2;
                X3 = Xde - A3*abs(C3*Xde - Pos(i));
                % new position = average of the three, kept within the duty limits
                Pos(i) = min(max((X1 + X2 + X3)/3, 0.31), Dmax);   % GWO lower bound = V_bat/V_oc ≈ 0.31
            end
            % serpentine order: alternate direction each iteration so the converter only
            % steps between neighbouring wolves (avoids large duty jumps and LC ringing)
            if mod(it, 2) == 1, Pos = sort(Pos, 'descend'); else, Pos = sort(Pos, 'ascend'); end
            idx = 1; Dc = Pos(1);
        end
    end

  % ================================================================================
  % STATE 3 - FLC FINE TRACKING
  % Normal operation. The fuzzy controller (outside this block) computes a small
  % duty step from dP/dV; this block just adds it and keeps D within the limits.
  %
  % Every sample the power is compared with the previous one (Eltamaly Eq. 13).
  % A jump of 5 % or more in a single 30 ms sample is too fast for the FLC's own
  % steps or for normal irradiance ramps, so it is treated as a shading change.
  % Modification: the jump must ALSO be at least DPMIN = 3.2 W. At low irradiance
  % (e.g. 15 W at 100 W/m^2) the FLC's own duty steps change P by more than 5 %,
  % but by only a few watts; without the floor they caused false restarts.
  % Pprev = 0 (set at handover) skips the comparison for one sample.
  %   config C -> start a full GWO search
  %   config D -> first try the stored peaks (state 4)
  % ================================================================================
  case 3
    if Pprev > 1 && abs(P - Pprev) >= EPS2*Pprev && abs(P - Pprev) >= DPMIN
        if useMem > 0.5 && memN > 0
            mi = 1; Dc = MemD(1); st = 4;     % test the most recent stored peak first
        else
            st = 1;
        end
    else
        Dc = min(max(Dc + dD_flc, Dmin), Dmax);
    end
    Pprev = P;

  % ================================================================================
  % STATE 4 - MEMORY CHECK (config D)
  % Each stored peak is tested for one sample. If the measured power is within 2 %
  % of the power stored with it, the same shading pattern has returned: stay at that
  % duty and hand straight to the FLC (a "hit", costing 1-3 evaluations instead of a
  % full search). If no stored peak matches (a "miss"), run a full GWO search, which
  % is seeded with the most recent stored peak in state 1.
  % ================================================================================
  case 4
    nEval = nEval + 1;
    if abs(P - MemP(mi)) <= TOLM*MemP(mi)
        Pprev = P; st = 3;                    % HIT
    else
        mi = mi + 1;
        if mi <= memN
            Dc = MemD(mi);                    % try the next stored peak
        else
            st = 1;                           % MISS -> seeded GWO search
        end
    end
end

% Outputs
D = Dc;  mode = st;  Xa = Xal;  nE = nEval;
end

% ----------------------------------------------------------------------------------
% Park-Miller pseudo-random number generator. Used instead of rand() so that the
% sequence is identical in every simulation (repeatable results) and works in
% Simulink code generation. Returns r in (0,1) and the updated seed s.
% ----------------------------------------------------------------------------------
function [r, s] = lcg(s)
s = mod(16807*s, 2147483647);
r = s/2147483647;
end
